simulink model "sim_DP2_2026_SFC_Nonlinear"  (R2025b)
settings: Solver=VariableStepAuto  StartTime=0.0  StopTime=Tsim  RelTol=1e-3
InitFcn:
  | myfile = 'sim_DP2_2026_SFC.p';
  | if exist(myfile, 'file')
  |     sim_DP2_2026_SFC
  | end
values from neighbouring files (symbols this model uses):
  A = [1 0 0 0 2.70127656662e-05 1.00008362958 0.0539210392304 0.167052905048 0.000996918625491 -3.04176177404e-06 0.993845368835 -0.00607175725634 ... (16 elements, 4x4)]    [Q2_Nonlinear_Workspace.mat]    (also in dp2_q1.m = sys_dt.A; dp2_q2_results.mat)
  a = 0.000406791666667    [Q2_Nonlinear_Workspace.mat]    (also in dp2_q1.m)
  B = [9.00986698557e-06 8.89404027496e-06 0.0179959975588 0.0177536761881]    [Q2_Nonlinear_Workspace.mat]    (also in dp2_q1.m = sys_dt.B; dp2_q2_results.mat)
  b = 0.000133128    [Q2_Nonlinear_Workspace.mat]    (also in dp2_q1.m)
  C = [1  0  0  0; 0  1  0  0]    [Q2_Nonlinear_Workspace.mat]    (also in dp2_q1.m = sys_dt.C; dp2_q2_results.mat)
  c = 0.00013158    [Q2_Nonlinear_Workspace.mat]    (also in dp2_q1.m)
  d = 0.00171    [Q2_Nonlinear_Workspace.mat]    (also in dp2_q1.m)
  Dp = 0.0005    [Q2_Nonlinear_Workspace.mat]    (also in dp2_q1.m)
  F = [-0.145177182245 15.3825401153 -0.458881050593 0.765291685949]    [Q2_Nonlinear_Workspace.mat]    (also in dp2_q2.m = place(A,B,pz); dp2_q2_results.mat; main_SFC.m = place(A,B,pz))
  h = 0.01518588    [Q2_Nonlinear_Workspace.mat]    (also in dp2_q1.m)
  kv = 0.005    [Q2_Nonlinear_Workspace.mat]    (also in dp2_q1.m)
  Lo = [0  0; 0  0; 0  0; 0  0]    [Q2_Nonlinear_Workspace.mat]    (also in main_SFC.m = place(A',C',po_z)')
  run_observer = 0    [Q2_Nonlinear_Workspace.mat]    (also in main_SFC.m = batch_case(2))
  ts = 0.001    [Q2_Nonlinear_Workspace.mat]    (also in dp2_q1.m; dp2_q2_results.mat)
  x_hat_o = [0 0 0 0]    [Q2_Nonlinear_Workspace.mat]    (also in main_SFC.m = [3*pi/180 -1*pi/180 0 0]')
settings Model: Creator=ricardoaguilera  LastModifiedBy=elinakim
settings SolverCC: AutoInsertRateTranBlk=on
settings DataIOCC: ReturnWorkspaceOutputs=off
settings DebuggingCC: AlgebraicLoopMsg=none

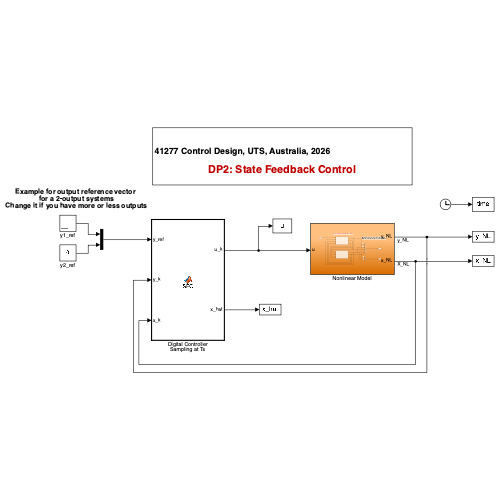
[thumbnail: Simulink's stored preview of the top-level diagram]
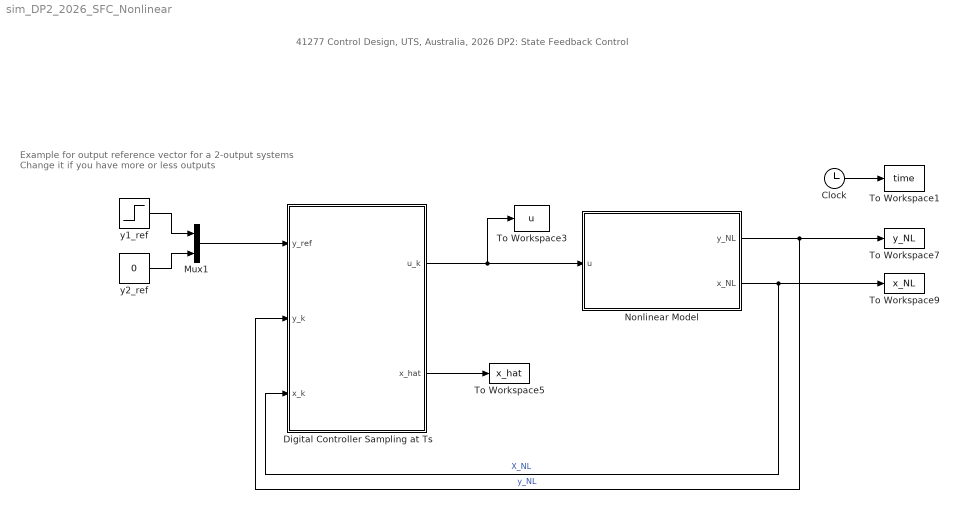
== system sim_DP2_2026_SFC_Nonlinear ==
  note: 41277 Control Design, UTS, Australia, 2026
      |
      | DP2: State Feedback Control
  note: Example for output reference vector
      | for a 2-output systems
      | Change it if you have more or less outputs
  Clock : Clock
  Digital Controller Sampling at Ts : MATLAB Function  TreatAsAtomicUnit=on  SystemSampleTime=ts
  Mux1 : Mux  Inputs=2
  Nonlinear Model : Subsystem
  To Workspace1 : ToWorkspace  VariableName=time  SampleTime=ts
  To Workspace3 : ToWorkspace  VariableName=u  SampleTime=ts
  To Workspace5 : ToWorkspace  VariableName=x_hat  SampleTime=ts
  To Workspace7 : ToWorkspace  VariableName=y_NL  SampleTime=ts
  To Workspace9 : ToWorkspace  VariableName=x_NL  SampleTime=ts
  y1_ref : Step  After=5*pi/180  SampleTime=0
  y2_ref : Constant  Value=0
  wires:
  Nonlinear Model/1(y_NL) -> Digital Controller Sampling at Ts/2(y_k), To Workspace7/1  "y_NL"
  y1_ref/1 -> Mux1/1
  y2_ref/1 -> Mux1/2
  Nonlinear Model/2(x_NL) -> Digital Controller Sampling at Ts/3(x_k), To Workspace9/1  "X_NL"
  Clock/1 -> To Workspace1/1
  Mux1/1 -> Digital Controller Sampling at Ts/1(y_ref)
  Digital Controller Sampling at Ts/1(u_k) -> To Workspace3/1, Nonlinear Model/1(u)
  Digital Controller Sampling at Ts/2(x_hat) -> To Workspace5/1

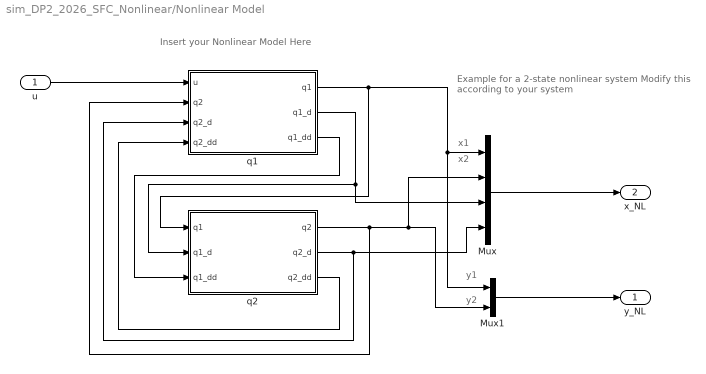
== system sim_DP2_2026_SFC_Nonlinear/Nonlinear Model ==
  note: x1
  note: Insert your Nonlinear Model Here
  note: x2
  note: y1
  note: y2
  note: Example for a 2-state nonlinear system
      | Modify this according to your system
  u : Inport
  Mux : Mux
  Mux1 : Mux  Inputs=2
  q1 : Subsystem
  q2 : Subsystem
  y_NL : Outport  VectorParamsAs1DForOutWhenUnconnected=off
  x_NL : Outport  Port=2  VectorParamsAs1DForOutWhenUnconnected=off
  wires:
  q2/3(q2_dd) -> q1/4(q2_dd)
  q2/2(q2_d) -> Mux/4, q1/3(q2_d)
  q2/1(q2) -> Mux/2, Mux1/2, q1/2(q2)
  q1/2(q1_d) -> Mux/3, q2/2(q1_d)
  q1/1(q1) -> q2/1(q1), Mux1/1, Mux/1
  Mux/1 -> x_NL/1
  Mux1/1 -> y_NL/1
  u/1 -> q1/1(u)
  q1/3(q1_dd) -> q2/3(q1_dd)

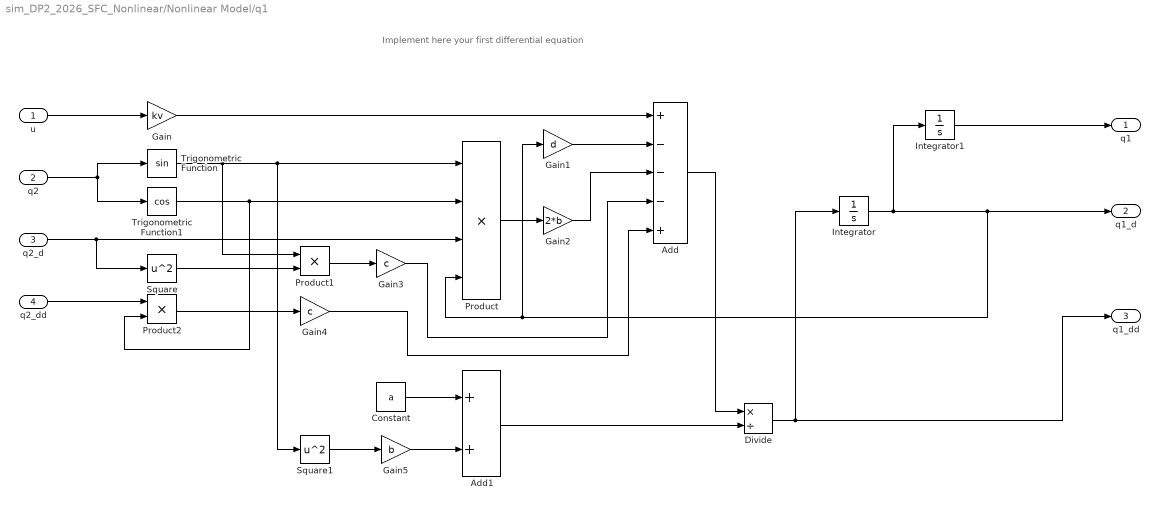
== system sim_DP2_2026_SFC_Nonlinear/Nonlinear Model/q1 ==
  note: Implement here your first differential equation
  u : Inport
  q2 : Inport  Port=2
  q2_d : Inport  Port=3
  q2_dd : Inport  Port=4
  Add : Sum  Inputs=+---+
  Add1 : Sum
  Constant : Constant  Value=a
  Divide : Product  Inputs=*/
  Gain : Gain  Gain=kv
  Gain1 : Gain  Gain=d
  Gain2 : Gain  Gain=2*b
  Gain3 : Gain  Gain=c
  Gain4 : Gain  Gain=c
  Gain5 : Gain  Gain=b
  Integrator : Integrator
  Integrator1 : Integrator
  Product : Product  Inputs=4
  Product1 : Product
  Product2 : Product
  Square : Math  Operator=square
  Square1 : Math  Operator=square
  Trigonometric Function : Trigonometry
  Trigonometric Function1 : Trigonometry  Operator=cos
  q1 : Outport  VectorParamsAs1DForOutWhenUnconnected=off
  q1_d : Outport  Port=2  VectorParamsAs1DForOutWhenUnconnected=off
  q1_dd : Outport  Port=3  VectorParamsAs1DForOutWhenUnconnected=off
  wires:
  Integrator/1 -> Gain1/1, Product/4, q1_d/1, Integrator1/1
  Integrator1/1 -> q1/1
  u/1 -> Gain/1
  q2/1 -> Trigonometric Function1/1, Trigonometric Function/1
  Trigonometric Function/1 -> Product/1, Square1/1, Product1/1
  Trigonometric Function1/1 -> Product2/2, Product/2
  q2_d/1 -> Square/1, Product/3
  Product/1 -> Gain2/1
  Square/1 -> Product1/2
  Product1/1 -> Gain3/1
  q2_dd/1 -> Product2/1
  Product2/1 -> Gain4/1
  Gain/1 -> Add/1
  Gain2/1 -> Add/3
  Gain3/1 -> Add/4
  Gain4/1 -> Add/5
  Square1/1 -> Gain5/1
  Add/1 -> Divide/1
  Add1/1 -> Divide/2
  Divide/1 -> Integrator/1, q1_dd/1
  Gain1/1 -> Add/2
  Gain5/1 -> Add1/2
  Constant/1 -> Add1/1

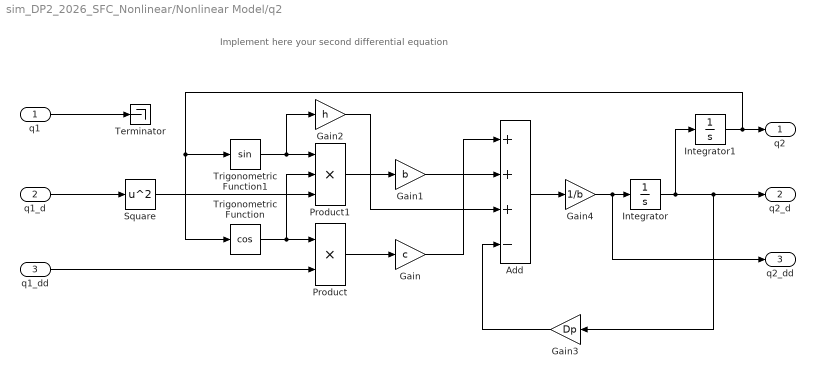
== system sim_DP2_2026_SFC_Nonlinear/Nonlinear Model/q2 ==
  note: Implement here your second differential equation
  q1 : Inport
  q1_d : Inport  Port=2
  q1_dd : Inport  Port=3
  Add : Sum  Inputs=+++-
  Gain : Gain  Gain=c
  Gain1 : Gain  Gain=b
  Gain2 : Gain  Gain=h
  Gain3 : Gain  Gain=Dp
  Gain4 : Gain  Gain=1/b
  Integrator : Integrator
  Integrator1 : Integrator
  Product : Product
  Product1 : Product  Inputs=3
  Square : Math  Operator=square
  Terminator : Terminator
  Trigonometric Function : Trigonometry  Operator=cos
  Trigonometric Function1 : Trigonometry
  q2 : Outport  VectorParamsAs1DForOutWhenUnconnected=off
  q2_d : Outport  Port=2  VectorParamsAs1DForOutWhenUnconnected=off
  q2_dd : Outport  Port=3  VectorParamsAs1DForOutWhenUnconnected=off
  wires:
  Integrator/1 -> Integrator1/1, Gain3/1, q2_d/1
  Integrator1/1 -> Trigonometric Function1/1, Trigonometric Function/1, q2/1
  q1/1 -> Terminator/1
  q1_dd/1 -> Product/2
  Trigonometric Function/1 -> Product1/2, Product/1
  Product/1 -> Gain/1
  q1_d/1 -> Square/1
  Trigonometric Function1/1 -> Gain2/1, Product1/1
  Product1/1 -> Gain1/1
  Square/1 -> Product1/3
  Gain/1 -> Add/1
  Gain1/1 -> Add/2
  Gain2/1 -> Add/3
  Gain3/1 -> Add/4
  Add/1 -> Gain4/1
  Gain4/1 -> q2_dd/1, Integrator/1

== matlab function sim_DP2_2026_SFC_Nonlinear/Digital Controller Sampling at Ts ==
  data: y_ref input; y_k input; x_k input; u_k output; F parameter; x_hat output; run_observer parameter; Lo parameter; A parameter; B parameter; C parameter; x_hat_o parameter
function [u_k, x_hat] = SFC(y_ref,y_k,x_k,F, ...
    run_observer,Lo,A,B,C,x_hat_o)

persistent x_hat_k

if isempty(x_hat_k)
    x_hat_k = x_hat_o;
end

x_hat = x_hat_k;

%% System size
n = size(A,1);
m = size(B,2);
p = size(C,1);

%% State references
x_ref = [y_ref(1); 0; 0; 0];
u_ref = 0;

u_k = zeros(m,1); % DO NOT DELETE

%% State-feedback control
if run_observer == 0
    u_k = -F*(x_k-x_ref) + u_ref;
else
    u_k = -F*(x_hat_k-x_ref) + u_ref;
end

%% Saturation: one motor, -10 V to +10 V
if u_k(1) > 10
    u_k(1) = 10;
elseif u_k(1) < -10
    u_k(1) = -10;
end

%% Observer
y_hat = C*x_hat_k;

x_hat_k = A*x_hat_k + B*u_k + Lo*(y_k-y_hat);

end
